simulink model "FCSMPC_double_vector_2025b"  (R2025b)
settings: Solver=FixedStepDiscrete  StartTime=0.0  StopTime=2  FixedStep=SimulinkTs  RelTol=1e-3
PreLoadFcn:
  | % Verzeichnis des Modells zum MATLAB-Pfad hinzufügen
  | modelDir = fileparts(get_param(bdroot, 'FileName'));
  | addpath(modelDir);
  | 
  | % Nur der Dateiname – kein Pfad!
  | set_param(bdroot, 'DataDictionary', 'FOC_params.sldd');
model workspace (MAT data in the model file):
  Np : Simulink.Parameter (value not decoded)
values from neighbouring files (symbols this model uses):
  Filter_Current_FilterTimeConst = 3.3333333333333335E-5    [FOC_params.sldd]
  Filter_Current_SensorTimeConst = 1.5915494309189535E-6    [FOC_params.sldd]
  FOC = evalin("base", "FOC")    [createFOC_SLDD.m]
  FOC_Control_Current_KIid = 10.0    [FOC_params.sldd]
  FOC_Control_Current_KIiq = 10.0    [FOC_params.sldd]
  FOC_Control_Current_KPid = 0.20418507462686566    [FOC_params.sldd]
  FOC_Control_Current_KPiq = 0.58674626865671642    [FOC_params.sldd]
  FOC_Control_Current_Krd = 0.8    [FOC_params.sldd]
  FOC_Control_Current_Krq = 0.8    [FOC_params.sldd]
  FOC_Control_Current_TclCur = 0.1    [FOC_params.sldd]
  FOC_Control_Current_Tnd = 0.1    [FOC_params.sldd]
  FOC_Control_Current_Tnq = 0.1    [FOC_params.sldd]
  FOC_Control_InverterVdc_V = 400.0    [FOC_params.sldd]
  FOC_Control_MotorImax_A = 650.0    [FOC_params.sldd]
  FOC_Control_MTPA_MTPV_nT_id_grid = -450.06704889786266 -439.56177000270145 -427.77784873303676 -416.66404703197372 -406.07553272717422 -395.15516533678584 -384.31176061747851 -374.03652088128132 -363.90551910193739 -353.79478643334204 -344.0221683092833 -334.51243453441936 -324.94614350292119 -315.21793409137081 -305.26543360965195 -295.21828280911944 -285.133916324101 -275.01232812136521 -264.86951532374729 -254.7797625148454 -244    [FOC_params.sldd]
  FOC_Control_MTPA_MTPV_nT_iq_grid = -449.09165648258488 -442.56958748923387 -437.25247759546528 -430.91792082419158 -423.83735797306491 -417.11730433547 -410.54064621830616 -403.71584331167304 -396.93611069310379 -390.15794305727007 -382.97216593027133 -375.44639668848538 -367.93447385667577 -360.57088856352266 -353.41289778449368 -346.34020584402072 -339.28416684923008 -332.22010880540631 -325.11927997033376 -317.92299905654966 -31    [FOC_params.sldd]
  FOC_Control_MTPA_MTPV_T_vec = -245.0 -240.0 -235.0 -230.0 -225.0 -220.0 -215.0 -210.0 -205.0 -200.0 -195.0 -190.0 -185.0 -180.0 -175.0 -170.0 -165.0 -160.0 -155.0 -150.0 -145.0 -140.0 -135.0 -130.0 -125.0 -120.0 -115.0 -110.0 -105.0 -100.0 -95.0 -90.0 -85.0 -80.0 -75.0 -70.0 -65.0 -60.0 -55.0 -50.0 -45.0 -40.0 -35.0 -30.0 -25.0 -20.0 -15.0 -10.0 -5.0 0.0 5.0 10.0 15.0 20.0 25.0 30.0 35.0 40.0 45.0 50.0 55.0 60.0 65.0 70.0 75.0    [FOC_params.sldd]
  FOC_Control_MTPA_MTPV_w_vec = 0.0 10.471975511965978 20.943951023931955 31.415926535897931 41.887902047863911 52.359877559829883 62.831853071795862 73.303828583761828 83.775804095727821 94.247779607693786 104.71975511965977 115.19173063162575 125.66370614359172 136.1356816555577 146.60765716752366 157.07963267948966 167.55160819145564 178.02358370342159 188.49555921538757 198.96753472735358 209.43951023931953 219.9114857512855    [FOC_params.sldd]
  FOC_Control_OpenLoop_Id_Ref_A = 0.0    [FOC_params.sldd]
  FOC_Control_OpenLoop_Iq_Ref_A = 0.0    [FOC_params.sldd]
  FOC_Control_OpenLoop_Ud_OpenLoop_V = 0.0    [FOC_params.sldd]
  FOC_Control_OpenLoop_Uq_OpenLoop_V = 0.0    [FOC_params.sldd]
  FOC_Control_RF_omegamech_rad_s = 3141.5926535897934    [FOC_params.sldd]
  FOC_Control_RF_RateCurrent_A = 500.0    [FOC_params.sldd]
  FOC_Control_RF_RateTrq_Nm = 500.0    [FOC_params.sldd]
  FOC_Control_theta_mechOffsetFix = 0.0    [FOC_params.sldd]
  FOC_Control_theta_mechOffsetTime = 0.0    [FOC_params.sldd]
  FOC_Control_TorqueRef_Nm = 10.0    [FOC_params.sldd]
  FOC_Control_Umax_V = 230.94010767585033    [FOC_params.sldd]
  FOC_Flag_ClosedLoopControl = 1.0    [FOC_params.sldd]
  FOC_Flag_ControlStrategy = 2.0    [FOC_params.sldd]
  FOC_Flag_PWMEnable = 1.0    [FOC_params.sldd]
  FOC_Flag_ResetControl = 0.0    [FOC_params.sldd]
  FOC_Flag_TorqueControl = 1.0    [FOC_params.sldd]
  FOC_LUT_DQLimiter_DQ_LUTScaling = 1.8749999999999995E-5    [FOC_params.sldd]
  FOC_PWM_AZSPWMMethod = 3.0    [FOC_params.sldd]
  FOC_PWM_HybridMode = 1.0    [FOC_params.sldd]
  FOC_PWM_LB1 = 0.5    [FOC_params.sldd]
  FOC_PWM_LB2 = 0.77    [FOC_params.sldd]
  FOC_PWM_PWMManuel = 1.0    [FOC_params.sldd]
  FOC_PWM_RSPWMMethod = 2.0    [FOC_params.sldd]
  FOC_PWM_UB1 = 0.66    [FOC_params.sldd]
  FOC_PWM_UB2 = 0.9    [FOC_params.sldd]
  FOC_SampleTime_TsCur = 0.0001    [FOC_params.sldd]
undefined symbols (not defined in the file or in its folder): dspblkCoreblockFVToolHelper, FCS, Filter, gcbh, Plant, SimulinkTs
libraries: hdlsllib x2, simulink x2, autolibfluxpmsm x1
(part 4 of 8)

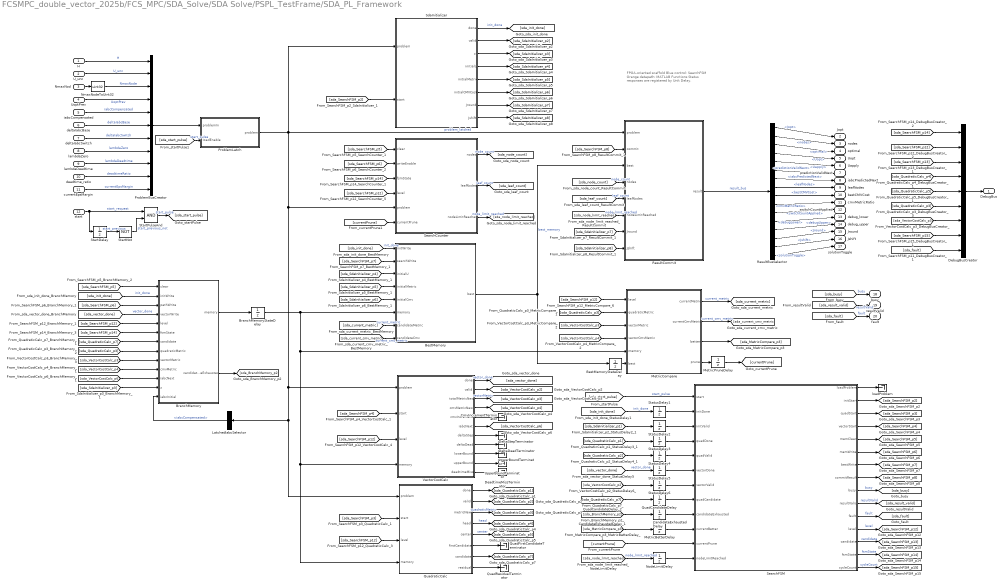
== system FCSMPC_double_vector_2025b/FCS_MPC/SDA_Solve/SDA Solve/PSPL_TestFrame/SDA_PL_Framework ==
  note: FPGA-oriented scaffold
      | Blue control: SearchFSM
      | Orange datapath: MATLAB Functions
      | Status responses are registered by Unit Delay.
  H : Inport
  U_unc : Inport  Port=2
  NmaxNod : Inport  Port=3
  UoptPrev : Inport  Port=4
  iabcCompensated : Inport  Port=5
  deltaIabcBase : Inport  Port=6
  deltaIabcSwitch : Inport  Port=7
  lambdaZero : Inport  Port=8
  lambdaDeadtime : Inport  Port=9
  deadtime_ratio : Inport  Port=10
  currentEpsMargin : Inport  Port=11
  start : Inport  Port=12  OutDataTypeStr=boolean
  BestMemory : MATLAB Function  TreatAsAtomicUnit=on
  BestMemoryStateDelay : UnitDelay  SampleTime=-1
  BranchMemory : MATLAB Function  TreatAsAtomicUnit=on
  BranchMemoryStateDelay : UnitDelay  SampleTime=-1
  CandidateExhaustedDelay : UnitDelay  InitialCondition=false  SampleTime=-1
  CmvIncrementTerminator : Terminator
  DeadtimeMissTerminator : Terminator
  DebugBusCreator : BusCreator  Inputs=9  OutDataTypeStr=Bus: SdaDebugBus
  DeltaDeadTerminator : Terminator
  DeltaStepTerminator : Terminator
  LatchedIabcSelector : BusSelector  OutputSignals=iabcCompensated
  LowerBoundTerminator : Terminator
  MetricBetterDelay : UnitDelay  InitialCondition=false  SampleTime=-1
  MetricCompare : MATLAB Function  TreatAsAtomicUnit=on
  MetricPruneDelay : UnitDelay  InitialCondition=false  SampleTime=-1
  NmaxNodeToUint32 : DataTypeConversion  OutDataTypeStr=uint32  SaturateOnIntegerOverflow=off  RndMeth=Floor
  NodeLimitDelay : UnitDelay  InitialCondition=false  SampleTime=-1
  ProblemBusCreator : BusCreator  Inputs=11  OutDataTypeStr=Bus: SdaProblemBus
  ProblemLatch : MATLAB Function  TreatAsAtomicUnit=on
  QuadCandidateDelay : UnitDelay  InitialCondition=false  SampleTime=-1
  QuadFirstCandidateTerminator : Terminator
  QuadResidualTerminator : Terminator
  QuadraticCalc : MATLAB Function  TreatAsAtomicUnit=on
  ResultBusSelector : BusSelector  OutputSignals=Jopt,nodes,optimal,Uopt,Uapply,predictionValidNext,iabcPredictedNext,leafNodes,bestCMVCost,cmvMetricRatio,switchCountApplied,debugLower,debugUpper,Jround,Jshift,solutionToggle
  ResultCommit : MATLAB Function  TreatAsAtomicUnit=on
  SdaInitializer : MATLAB Function  TreatAsAtomicUnit=on
  SearchCounter : MATLAB Function  TreatAsAtomicUnit=on
  SearchFSM : Stateflow chart  TreatAsAtomicUnit=on
  StartDelay : UnitDelay  InitialCondition=false  SampleTime=-1  HasFrameUpgradeWarning=on
  StartNot : Logic  Operator=NOT  AllPortsSameDT=off  OutDataTypeStr=boolean
  StartPulseAnd : Logic  AllPortsSameDT=off  OutDataTypeStr=boolean
  StatusDelay{1..6} (6 alike) : UnitDelay  InitialCondition=false  SampleTime=-1
  UpperBoundTerminator : Terminator
  VectorCostCalc : MATLAB Function  TreatAsAtomicUnit=on
  loadProblem : Terminator
  DebugBus : Outport  OutDataTypeStr=Bus: SdaDebugBus
  Jopt : Outport  Port=2
  nodes : Outport  Port=3
  optimal : Outport  Port=4
  Uopt : Outport  Port=5
  Uapply : Outport  Port=6
  predictionValidNext : Outport  Port=7
  iabcPredictedNext : Outport  Port=8
  leafNodes : Outport  Port=9
  bestCMVCost : Outport  Port=10
  cmvMetricRatio : Outport  Port=11
  switchCountApplied : Outport  Port=12
  debug_lower : Outport  Port=13
  debug_upper : Outport  Port=14
  Jround : Outport  Port=15
  Jshift : Outport  Port=16
  solutionToggle : Outport  Port=17
  busy : Outport  Port=18
  resultValid : Outport  Port=19
  fault : Outport  Port=20
  wires:
  NodeLimitDelay/1 -> SearchFSM/12(nodeLimitReached)
  MetricPruneDelay/1 -> [currentPrune]
  MetricBetterDelay/1 -> SearchFSM/10(currentBetter)
  BestMemoryStateDelay/1 -> MetricCompare/6(best)
  CandidateExhaustedDelay/1 -> SearchFSM/9(candidateExhausted)
  QuadCandidateDelay/1 -> SearchFSM/8(quadCandidate)
  BranchMemoryStateDelay/1 -> QuadraticCalc/4(memory), VectorCostCalc/4(memory), MetricCompare/5(memory), BestMemory/6(memory)
  NmaxNodeToUint32/1 -> ProblemBusCreator/3  "NmaxNode"
  NmaxNod/1 -> NmaxNodeToUint32/1
  DebugBusCreator/1 -> DebugBus/1
  SearchFSM/11(fault) -> [sda_fault]  "fault"
  StatusDelay6/1 -> SearchFSM/7(vectorValid)
  StatusDelay5/1 -> SearchFSM/6(vectorDone)
  StatusDelay4/1 -> SearchFSM/5(quadValid)
  StatusDelay3/1 -> SearchFSM/4(quadDone)
  StatusDelay2/1 -> SearchFSM/3(initValid)
  StatusDelay1/1 -> SearchFSM/2(initDone)
  ProblemBusCreator/1 -> ProblemLatch/1(problemIn)
  currentEpsMargin/1 -> ProblemBusCreator/11  "currentEpsMargin"
  deadtime_ratio/1 -> ProblemBusCreator/10  "deadtimeRatio"
  lambdaDeadtime/1 -> ProblemBusCreator/9  "lambdaDeadtime"
  lambdaZero/1 -> ProblemBusCreator/8  "lambdaZero"
  deltaIabcSwitch/1 -> ProblemBusCreator/7  "deltaIabcSwitch"
  deltaIabcBase/1 -> ProblemBusCreator/6  "deltaIabcBase"
  iabcCompensated/1 -> ProblemBusCreator/5  "iabcCompensated"
  UoptPrev/1 -> ProblemBusCreator/4  "UoptPrev"
  U_unc/1 -> ProblemBusCreator/2  "U_unc"
  H/1 -> ProblemBusCreator/1  "H"
  start/1 -> StartDelay/1, StartPulseAnd/1  "start_request"
  StartDelay/1 -> StartNot/1  "start_previous"
  StartNot/1 -> StartPulseAnd/2  "start_previous_not"
  StartPulseAnd/1 -> [sda_start_pulse]  "start_pulse"
  [sda_start_pulse] -> SearchFSM/1(start)  "start_pulse"
  ResultBusSelector/1 -> Jopt/1  "<Jopt>"
  ResultBusSelector/2 -> nodes/1  "<nodes>"
  ResultBusSelector/3 -> optimal/1  "<optimal>"
  ResultBusSelector/4 -> Uopt/1  "<Uopt>"
  ResultBusSelector/5 -> Uapply/1  "<Uapply>"
  ResultBusSelector/6 -> predictionValidNext/1  "<predictionValidNext>"
  ResultBusSelector/7 -> iabcPredictedNext/1  "<iabcPredictedNext>"
  ResultBusSelector/8 -> leafNodes/1  "<leafNodes>"
  ResultBusSelector/9 -> bestCMVCost/1  "<bestCMVCost>"
  ResultBusSelector/10 -> cmvMetricRatio/1  "<cmvMetricRatio>"
  ResultBusSelector/11 -> switchCountApplied/1  "<switchCountApplied>"
  ResultBusSelector/12 -> debug_lower/1  "<debugLower>"
  ResultBusSelector/13 -> debug_upper/1  "<debugUpper>"
  ResultBusSelector/14 -> Jround/1  "<Jround>"
  ResultBusSelector/15 -> Jshift/1  "<Jshift>"
  ResultBusSelector/16 -> solutionToggle/1  "<solutionToggle>"
  SearchFSM/9(busy) -> [sda_busy]  "busy"
  [sda_busy] -> busy/1  "busy"
  SearchFSM/10(resultValid) -> [sda_result_valid]  "resultValid"
  [sda_result_valid] -> resultValid/1  "resultValid"
  [sda_fault] -> fault/1  "fault"
  ProblemLatch/1(problem) -> QuadraticCalc/1(problem), LatchedIabcSelector/1, VectorCostCalc/1(problem), SearchCounter/5(problem), ResultCommit/1(problem), SdaInitializer/1(problem)  "problem_latched"
  BestMemory/1(best) -> ResultCommit/3(best), BestMemoryStateDelay/1  "best_memory"
  ResultCommit/1(result) -> ResultBusSelector/1  "result_bus"
  SdaInitializer/1(done) -> [sda_init_done]  "init_done"
  [sda_init_done] -> StatusDelay1/1  "init_done"
  [sda_init_done] -> BranchMemory/2(initWrite)  "init_done"
  [sda_init_done] -> BestMemory/1(initWrite)  "init_done"
  VectorCostCalc/1(done) -> [sda_vector_done]  "vector_done"
  [sda_vector_done] -> BranchMemory/4(vectorWrite)  "vector_done"
  [sda_vector_done] -> StatusDelay5/1  "vector_done"
  MetricCompare/1(currentMetric) -> [sda_current_metric]  "current_metric"
  [sda_current_metric] -> BestMemory/7(candidateMetric)  "current_metric"
  MetricCompare/2(currentCmvMetric) -> [sda_current_cmv_metric]  "current_cmv_metric"
  [sda_current_cmv_metric] -> BestMemory/8(candidateCmv)  "current_cmv_metric"
  SearchCounter/1(nodes) -> [sda_node_count]  "node_count"
  [sda_node_count] -> ResultCommit/4(nodes)  "node_count"
  SearchCounter/2(leafNodes) -> [sda_leaf_count]  "leaf_count"
  [sda_leaf_count] -> ResultCommit/5(leafNodes)  "leaf_count"
  SearchCounter/3(nodeLimitReached) -> [sda_node_limit_reached]  "node_limit_reached"
  [sda_node_limit_reached] -> ResultCommit/6(nodeLimitReached)  "node_limit_reached"
  [sda_node_limit_reached] -> NodeLimitDelay/1  "node_limit_reached"
  SearchFSM/1(loadProblem) -> loadProblem/1
  SearchFSM/2(initStart) -> [sda_SearchFSM_p2]
  [sda_SearchFSM_p2] -> SdaInitializer/2(start)
  SearchFSM/3(quadStart) -> [sda_SearchFSM_p3]
  [sda_SearchFSM_p3] -> QuadraticCalc/2(start)
  SearchFSM/4(vectorStart) -> [sda_SearchFSM_p4]
  [sda_SearchFSM_p4] -> VectorCostCalc/2(start)
  SearchFSM/5(memClear) -> [sda_SearchFSM_p5]
  [sda_SearchFSM_p5] -> SearchCounter/1(clear)
  [sda_SearchFSM_p5] -> BranchMemory/1(clear)
  SearchFSM/6(memWrite) -> [sda_SearchFSM_p6]
  [sda_SearchFSM_p6] -> BranchMemory/3(pathWrite)
  [sda_SearchFSM_p6] -> SearchCounter/2(writeEnable)
  SearchFSM/7(bestWrite) -> [sda_SearchFSM_p7]
  [sda_SearchFSM_p7] -> BestMemory/2(searchWrite)
  SearchFSM/8(commitResult) -> [sda_SearchFSM_p8]
  [sda_SearchFSM_p8] -> ResultCommit/2(commit)
  [sda_fault] -> DebugBusCreator/9
  SearchFSM/12(level) -> [sda_SearchFSM_p12]  "level"
  [sda_SearchFSM_p12] -> BranchMemory/5(level)
  [sda_SearchFSM_p12] -> DebugBusCreator/2
  [sda_SearchFSM_p12] -> QuadraticCalc/3(level)
  [sda_SearchFSM_p12] -> VectorCostCalc/3(level)
  [sda_SearchFSM_p12] -> SearchCounter/4(level)
  [sda_SearchFSM_p12] -> MetricCompare/1(level)
  SearchFSM/13(candidate) -> [sda_SearchFSM_p13]  "candidate"
  [sda_SearchFSM_p13] -> DebugBusCreator/3
  SearchFSM/14(fsmState) -> [sda_SearchFSM_p14]  "fsmState"
  [sda_SearchFSM_p14] -> SearchCounter/3(fsmState)
  [sda_SearchFSM_p14] -> DebugBusCreator/1
  [sda_SearchFSM_p14] -> BranchMemory/6(fsmState)
  SearchFSM/15(cycleCount) -> [sda_SearchFSM_p15]  "cycleCount"
  [sda_SearchFSM_p15] -> DebugBusCreator/8
  SdaInitializer/2(valid) -> [sda_SdaInitializer_p2]
  [sda_SdaInitializer_p2] -> StatusDelay2/1
  SdaInitializer/3(z) -> [sda_SdaInitializer_p3]
  [sda_SdaInitializer_p3] -> BranchMemory/12(z)
  SdaInitializer/4(initialU) -> [sda_SdaInitializer_p4]
  [sda_SdaInitializer_p4] -> BestMemory/3(initialU)
  SdaInitializer/5(initialMetric) -> [sda_SdaInitializer_p5]
  [sda_SdaInitializer_p5] -> BestMemory/4(initialMetric)
  SdaInitializer/6(initialCMVCost) -> [sda_SdaInitializer_p6]
  [sda_SdaInitializer_p6] -> BestMemory/5(initialCmv)
  SdaInitializer/7(Jround) -> [sda_SdaInitializer_p7]
  [sda_SdaInitializer_p7] -> ResultCommit/7(Jround)
  SdaInitializer/8(Jshift) -> [sda_SdaInitializer_p8]
  [sda_SdaInitializer_p8] -> ResultCommit/8(Jshift)
  QuadraticCalc/1(done) -> [sda_QuadraticCalc_p1]
  [sda_QuadraticCalc_p1] -> StatusDelay3/1
  QuadraticCalc/2(valid) -> [sda_QuadraticCalc_p2]
  [sda_QuadraticCalc_p2] -> StatusDelay4/1
  QuadraticCalc/3(metricNew) -> [sda_QuadraticCalc_p3]  "quadraticMetric"
  [sda_QuadraticCalc_p3] -> MetricCompare/2(quadraticMetric)
  [sda_QuadraticCalc_p3] -> BranchMemory/8(quadraticMetric)
  [sda_QuadraticCalc_p3] -> DebugBusCreator/6
  QuadraticCalc/4(head) -> [sda_QuadraticCalc_p4]  "head"
  [sda_QuadraticCalc_p4] -> DebugBusCreator/4
  QuadraticCalc/5(center) -> [sda_QuadraticCalc_p5]  "center"
  [sda_QuadraticCalc_p5] -> DebugBusCreator/5
  QuadraticCalc/6(firstCandidate) -> QuadFirstCandidateTerminator/1
  QuadraticCalc/7(candidate) -> [sda_QuadraticCalc_p7]
  [sda_QuadraticCalc_p7] -> BranchMemory/7(candidate)
  [sda_QuadraticCalc_p7] -> QuadCandidateDelay/1
  QuadraticCalc/8(residual) -> QuadResidualTerminator/1
  VectorCostCalc/2(valid) -> [sda_VectorCostCalc_p2]
  [sda_VectorCostCalc_p2] -> StatusDelay6/1
  VectorCostCalc/3(totalMetricNew) -> [sda_VectorCostCalc_p3]  "vectorMetric"
  [sda_VectorCostCalc_p3] -> DebugBusCreator/7
  [sda_VectorCostCalc_p3] -> MetricCompare/3(vectorMetric)
  [sda_VectorCostCalc_p3] -> BranchMemory/9(vectorMetric)
  VectorCostCalc/4(cmvMetricNew) -> [sda_VectorCostCalc_p4]
  [sda_VectorCostCalc_p4] -> BranchMemory/10(cmvMetric)
  [sda_VectorCostCalc_p4] -> MetricCompare/4(vectorCmvMetric)
  VectorCostCalc/5(cmvIncrement) -> CmvIncrementTerminator/1
  VectorCostCalc/6(iabcNext) -> [sda_VectorCostCalc_p6]
  [sda_VectorCostCalc_p6] -> BranchMemory/11(iabcNext)
  VectorCostCalc/7(deltaStep) -> DeltaStepTerminator/1
  VectorCostCalc/8(deltaDead) -> DeltaDeadTerminator/1
  VectorCostCalc/9(lowerBound) -> LowerBoundTerminator/1
  VectorCostCalc/10(upperBound) -> UpperBoundTerminator/1
  VectorCostCalc/11(deadtimeMiss) -> DeadtimeMissTerminator/1
  BranchMemory/1(memory) -> BranchMemoryStateDelay/1
  BranchMemory/2(candidateExhausted) -> [sda_BranchMemory_p2]
  [sda_BranchMemory_p2] -> CandidateExhaustedDelay/1
  MetricCompare/3(better) -> [sda_MetricCompare_p3]
  [sda_MetricCompare_p3] -> MetricBetterDelay/1
  MetricCompare/4(prune) -> MetricPruneDelay/1
  [currentPrune] -> SearchFSM/11(currentPrune)
  [currentPrune] -> SearchCounter/6(currentPrune)
  LatchedIabcSelector/1 -> BranchMemory/13(iabcInitial)  "<iabcCompensated>"
  [sda_start_pulse] -> ProblemLatch/2(loadEnable)  "start_pulse"

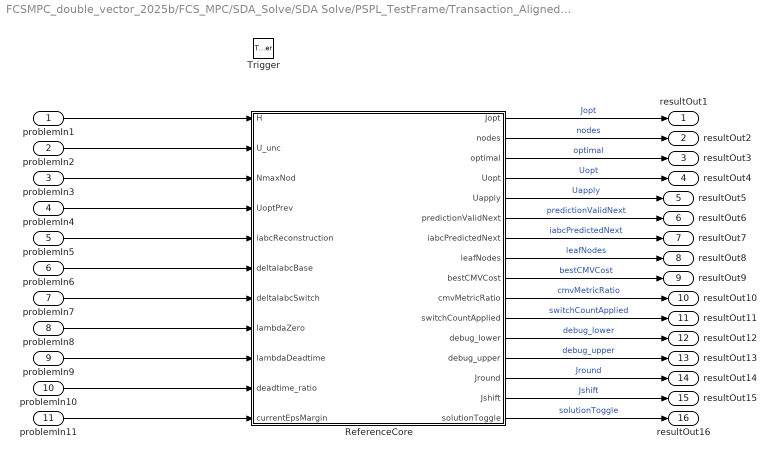
== system FCSMPC_double_vector_2025b/FCS_MPC/SDA_Solve/SDA Solve/PSPL_TestFrame/Transaction_Aligned_Reference ==
  problemIn1 : Inport
  problemIn2 : Inport  Port=2
  problemIn3 : Inport  Port=3
  problemIn4 : Inport  Port=4
  problemIn5 : Inport  Port=5
  problemIn6 : Inport  Port=6
  problemIn7 : Inport  Port=7
  problemIn8 : Inport  Port=8
  problemIn9 : Inport  Port=9
  problemIn10 : Inport  Port=10
  problemIn11 : Inport  Port=11
  Trigger : TriggerPort  VariantControl=(inherit)
  ReferenceCore : MATLAB Function  TreatAsAtomicUnit=on
  resultOut1 : Outport
  resultOut2 : Outport  Port=2
  resultOut3 : Outport  Port=3
  resultOut4 : Outport  Port=4
  resultOut5 : Outport  Port=5
  resultOut6 : Outport  Port=6
  resultOut7 : Outport  Port=7
  resultOut8 : Outport  Port=8
  resultOut9 : Outport  Port=9
  resultOut10 : Outport  Port=10
  resultOut11 : Outport  Port=11
  resultOut12 : Outport  Port=12
  resultOut13 : Outport  Port=13
  resultOut14 : Outport  Port=14
  resultOut15 : Outport  Port=15
  resultOut16 : Outport  Port=16
  wires:
  problemIn1/1 -> ReferenceCore/1(H)
  problemIn2/1 -> ReferenceCore/2(U_unc)
  problemIn3/1 -> ReferenceCore/3(NmaxNod)
  problemIn4/1 -> ReferenceCore/4(UoptPrev)
  problemIn5/1 -> ReferenceCore/5(iabcReconstruction)
  problemIn6/1 -> ReferenceCore/6(deltaIabcBase)
  problemIn7/1 -> ReferenceCore/7(deltaIabcSwitch)
  problemIn8/1 -> ReferenceCore/8(lambdaZero)
  problemIn9/1 -> ReferenceCore/9(lambdaDeadtime)
  problemIn10/1 -> ReferenceCore/10(deadtime_ratio)
  problemIn11/1 -> ReferenceCore/11(currentEpsMargin)
  ReferenceCore/1(Jopt) -> resultOut1/1  "Jopt"
  ReferenceCore/2(nodes) -> resultOut2/1  "nodes"
  ReferenceCore/3(optimal) -> resultOut3/1  "optimal"
  ReferenceCore/4(Uopt) -> resultOut4/1  "Uopt"
  ReferenceCore/5(Uapply) -> resultOut5/1  "Uapply"
  ReferenceCore/6(predictionValidNext) -> resultOut6/1  "predictionValidNext"
  ReferenceCore/7(iabcPredictedNext) -> resultOut7/1  "iabcPredictedNext"
  ReferenceCore/8(leafNodes) -> resultOut8/1  "leafNodes"
  ReferenceCore/9(bestCMVCost) -> resultOut9/1  "bestCMVCost"
  ReferenceCore/10(cmvMetricRatio) -> resultOut10/1  "cmvMetricRatio"
  ReferenceCore/11(switchCountApplied) -> resultOut11/1  "switchCountApplied"
  ReferenceCore/12(debug_lower) -> resultOut12/1  "debug_lower"
  ReferenceCore/13(debug_upper) -> resultOut13/1  "debug_upper"
  ReferenceCore/14(Jround) -> resultOut14/1  "Jround"
  ReferenceCore/15(Jshift) -> resultOut15/1  "Jshift"
  ReferenceCore/16(solutionToggle) -> resultOut16/1  "solutionToggle"

== stateflow chart FCSMPC_double_vector_2025b/FCS_MPC/CurrentRefCalc/Current_RateLimiter/RateLimiter1 ==
  settings: updateMethod=DISCRETE  sampleTime=FOC.SampleTime.TsSpeed
  state IDLE
  state Rising
    entry:  y =  fi(y_prev +dT * R, 1, 32, 18);
    exit: y_prev = y;
  state Falling
    entry:  y = fi(y_prev+dT * F, 1, 32, 18);
    exit: y_prev = y;
  state Directpassage
    entry:  y = u;
    exit: y_prev = y;
  (default) -> IDLE
  IDLE -> (junction 22)
  (junction 22) -> Rising [order 1] : [(u-y_prev)/dT>=R]
  (junction 22) -> Falling [order 2] : [(u-y_prev)/dT<=F]
  Rising -> (junction 22)
  Falling -> (junction 22)
  Directpassage -> (junction 22)
  (junction 22) -> Directpassage [order 3] : [(u-y_prev)/dT<R && (u-y_prev)/dT>F]
  data: u input fixdt(1,32,18); R input fixdt(1,32,18); F input fixdt(1,32,18); dT constant fixdt(1,32,18) size=1 =FOC.SampleTime.TsSpeed; y output fixdt(1,32,18); y_prev local fixdt(1,32,18) =0

== stateflow chart FCSMPC_double_vector_2025b/FCS_MPC/CurrentRefCalc/RateLimiter ==
  settings: updateMethod=DISCRETE  sampleTime=FOC.SampleTime.TsSpeed
  state IDLE
  state Rising
    entry:  y =  fi(y_prev +dT * R, 1, 32, 18);
    exit: y_prev = y;
  state Falling
    entry:  y = fi(y_prev+dT * F, 1, 32, 18);
    exit: y_prev = y;
  state Directpassage
    entry:  y = u;
    exit: y_prev = y;
  (default) -> IDLE
  IDLE -> (junction 22)
  (junction 22) -> Rising [order 1] : [(u-y_prev)/dT>=R]
  (junction 22) -> Falling [order 2] : [(u-y_prev)/dT<=F]
  Rising -> (junction 22)
  Falling -> (junction 22)
  Directpassage -> (junction 22)
  (junction 22) -> Directpassage [order 3] : [(u-y_prev)/dT<R && (u-y_prev)/dT>F]
  data: u input fixdt(1,32,18); R input fixdt(1,32,18); F input fixdt(1,32,18); dT constant fixdt(1,32,18) size=1 =FOC.SampleTime.TsSpeed; y output fixdt(1,32,18); y_prev local fixdt(1,32,18) =0

== matlab function FCSMPC_double_vector_2025b/FCS_MPC/SDA_Solve/SDA Solve/PSPL_TestFrame/SDA_PL_Framework/BestMemory ==
  data: initWrite input boolean size=[1 1]; searchWrite input boolean size=[1 1]; best output Bus: SdaBestBus size=[1 1]; initialU input double size=[15 1]; initialMetric input double size=[1 1]; initialCmv input double size=[1 1]; memory input Bus: SdaMemoryBus size=[1 1]; candidateMetric input double size=[1 1]; candidateCmv input double size=[1 1]
function best = BestMemory(initWrite,searchWrite,initialU,initialMetric,initialCmv,memory,candidateMetric,candidateCmv)
%#codegen
persistent state
if isempty(state)
 state.bestU=false(15,1); state.bestMetric=realmax;
 state.bestCMVCost=0.0; state.bestValid=false;
end
if initWrite
 state.bestU=initialU>0.5; state.bestMetric=initialMetric;
 state.bestCMVCost=initialCmv; state.bestValid=isfinite(initialMetric);
elseif searchWrite&&candidateMetric<state.bestMetric
 state.bestU=memory.Uwork; state.bestMetric=candidateMetric;
 state.bestCMVCost=candidateCmv; state.bestValid=isfinite(candidateMetric);
end
best=state;
end

== stateflow chart FCSMPC_double_vector_2025b/Plant_PMSM_INV/RateLimiter ==
  settings: updateMethod=DISCRETE  sampleTime=FOC.SampleTime.TsSpeed
  state IDLE
  state Rising
    entry:  y = dT*R+y_prev;
    exit: y_prev = y;
  state Falling
    entry:  y = dT*F+y_prev;
    exit: y_prev = y;
  state Directpassage
    entry:  y = u;
    exit: y_prev = y;
  (default) -> IDLE
  IDLE -> (junction 22)
  (junction 22) -> Rising [order 1] : [(u-y_prev)/dT>=R]
  (junction 22) -> Falling [order 2] : [(u-y_prev)/dT<=F]
  Rising -> (junction 22)
  Falling -> (junction 22)
  Directpassage -> (junction 22)
  (junction 22) -> Directpassage [order 3] : [(u-y_prev)/dT<R && (u-y_prev)/dT>F]
  data: u input; R input; F input; dT constant double size=1 =FOC.SampleTime.TsSpeed; y output; y_prev local double =0

== matlab function FCSMPC_double_vector_2025b/FCS_MPC/SDA_Solve/SDA Solve/PSPL_TestFrame/Transaction_Aligned_Reference/ReferenceCore ==
  data: H input double size=[15 15]; Jopt output double size=[1 1]; U_unc input double size=[15 1]; NmaxNod input double size=[1 1]; UoptPrev input double size=[15 1]; iabcReconstruction input double size=[3 1]; deltaIabcBase input double size=[3 1]; deltaIabcSwitch input double size=[3 3]; lambdaZero input double size=[1 1]; lambdaDeadtime input double size=[1 1]; deadtime_ratio input double size=[1 1]; currentEpsMargin input double size=[1 1]; nodes output double size=[1 1]; optimal output boolean size=[1 1]; Uopt output double size=[15 1]; Uapply output double size=[6 1]; predictionValidNext output boolean size=[1 1]; iabcPredictedNext output double size=[3 1]; leafNodes output double size=[1 1]; bestCMVCost output double size=[1 1]; cmvMetricRatio output double size=[1 1]; switchCountApplied output double size=[1 1]; debug_lower output double size=[3 1]; debug_upper output double size=[3 1]; Jround output double size=[1 1]; Jshift output double size=[1 1]; solutionToggle output boolean size=[1 1]
function [Jopt, nodes, optimal, Uopt, Uapply, ...
    predictionValidNext,iabcPredictedNext, ...
    leafNodes, bestCMVCost, cmvMetricRatio, switchCountApplied, ...
    debug_lower, debug_upper, Jround, Jshift, solutionToggle] = ...
    SDA_Solve_Synchronized(H, U_unc, NmaxNod, UoptPrev, ...
    iabcReconstruction, deltaIabcBase, deltaIabcSwitch, ...
    lambdaZero, lambdaDeadtime, deadtime_ratio, currentEpsMargin)
%SDA_SOLVE Independent double-vector SDA MATLAB Function module.
% The first five ports follow FCSMPC_IdealSDA. Feed Uopt back to UoptPrev
% through a Unit Delay initialized with zeros(15,1). UapplyFirst and
% UapplySecond are applied successively for half an external period each.

Np = 5;
nu = 3;
n = numel(U_unc);

Ubar = H*U_unc;
uprev = UoptPrev(4:6);
deadtimeRatio = deadtime_ratio;

Uround = min(max(round(U_unc),0.0),1.0);
Ushift = zeros(n,1);
Ushift(1:n-nu) = UoptPrev(nu+1:n);
Ushift(n-nu+1:n) = UoptPrev(n-nu+1:n);
Jround = norm(H*(Uround-U_unc),2)^2;
Jshift = norm(H*(Ushift-U_unc),2)^2;
if Jshift < Jround
    Uini = Ushift;
else
    Uini = Uround;
end

bestCMVCost = sequence_cmv_cost_predicted( ...
    Uini,uprev,iabcReconstruction,Np,nu, ...
    deltaIabcBase,deltaIabcSwitch,lambdaZero,lambdaDeadtime, ...
    deadtimeRatio,currentEpsMargin);
bestMetric = norm(H*(Uini-U_unc),2)^2+bestCMVCost;
Uopt = Uini;

U = zeros(n,1);
kidx = ones(n,1);
d2s = zeros(n+1,1);
cmvD2s = zeros(n+1,1);
iabcPrediction = zeros(3,Np+1);
iabcPrediction(:,1) = iabcReconstruction;
nodes = 0;
leafNodes = 0;
optimal = true;
i = 1;

while i >= 1
    if kidx(i) > 2
        kidx(i) = 1;
        i = i-1;
        continue;
    end
    head = 0.0;
    if i > 1
        head = H(i,1:i-1)*U(1:i-1);
    end
    center = (Ubar(i)-head)/H(i,i);
    if center <= 0.5
        firstCandidate = 0.0;
    else
        firstCandidate = 1.0;
    end
    if kidx(i) == 1
        candidate = firstCandidate;
    else
        candidate = 1.0-firstCandidate;
    end
    kidx(i) = kidx(i)+1;
    U(i) = candidate;
    nodes = nodes+1;
    if NmaxNod > 0 && nodes > NmaxNod
        optimal = false;
        break;
    end

    residual = Ubar(i)-head-H(i,i)*candidate;
    metricNew = d2s(i)+residual*residual;
    cmvMetricNew = cmvD2s(i);
    if mod(i,nu) == 0
        predictionStep = i/nu;
        blockStart = i-nu+1;
        uCurrent = U(blockStart:i);
        if predictionStep == 1
            uPrevious = uprev;
        else
            uPrevious = U(blockStart-nu:blockStart-1);
        end
        iabcBeforeSwitch = iabcPrediction(:,predictionStep);
        [deltaStep,deltaDead] = deadtime_corrected_current_step( ...
            uPrevious,uCurrent,iabcBeforeSwitch, ...
            deltaIabcBase,deltaIabcSwitch,deadtimeRatio,currentEpsMargin);
        cmvIncrement = cmv_cost( ...
            uPrevious,uCurrent,iabcBeforeSwitch,deltaDead, ...
            lambdaZero,lambdaDeadtime,currentEpsMargin);
        metricNew = metricNew+cmvIncrement;
        cmvMetricNew = cmvMetricNew+cmvIncrement;
        iabcPrediction(:,predictionStep+1) = iabcBeforeSwitch+deltaStep;
    end
    if metricNew > bestMetric
        continue;
    end
    if i == n
        leafNodes = leafNodes+1;
        if metricNew < bestMetric
            bestMetric = metricNew;
            Uopt = U;
            bestCMVCost = cmvMetricNew;
        end
    else
        d2s(i+1) = metricNew;
        cmvD2s(i+1) = cmvMetricNew;
        i = i+1;
        kidx(i) = 1;
    end
end

if ~isfinite(bestMetric)
    Uopt = repmat(uprev,Np,1);
end

Uapply = Uopt(1:6);
UapplyFirst = Uopt(1:3);
UapplySecond = Uopt(4:6);

[deltaFirst,~] = deadtime_corrected_current_step( ...
    uprev,UapplyFirst,iabcReconstruction, ...
    deltaIabcBase,deltaIabcSwitch, ...
    deadtimeRatio,currentEpsMargin);
iabcAfterFirst = iabcReconstruction + deltaFirst;

[deltaSecond,~] = deadtime_corrected_current_step( ...
    UapplyFirst,UapplySecond,iabcAfterFirst, ...
    deltaIabcBase,deltaIabcSwitch,deadtimeRatio,currentEpsMargin);
iabcPredictedNext = iabcAfterFirst+deltaSecond;

switchCountApplied = sum(abs(UapplyFirst-uprev))+ ...
    sum(abs(UapplySecond-UapplyFirst));
Jopt = bestMetric;
if Jopt > eps
    cmvMetricRatio = bestCMVCost/Jopt;
else
    cmvMetricRatio = 0.0;
end
[~,debugDeltaDead] = deadtime_corrected_current_step( ...
    uprev,UapplyFirst,iabcReconstruction,deltaIabcBase,deltaIabcSwitch, ...
    deadtimeRatio,currentEpsMargin);
[~,debug_lower,debug_upper] = cmv_cost( ...
    uprev,UapplyFirst,iabcReconstruction,debugDeltaDead, ...
    lambdaZero,lambdaDeadtime,currentEpsMargin);
predictionValidNext = true;

% Toggle once after every completed SDA solution. The downstream switch
% detects this edge and explicitly restarts from the first vector.
persistent solutionToggleState
if isempty(solutionToggleState)
    solutionToggleState = false;
end
solutionToggleState = ~solutionToggleState;
solutionToggle = solutionToggleState;
end

function [deltaStep,deltaDead] = deadtime_corrected_current_step( ...
    uPrevious,uCurrent,iabcBeforeSwitch, ...
    deltaBase,deltaSwitch,deadtimeRatio,currentEps)
uDead = uCurrent;
changed = (uPrevious ~= uCurrent);
signEps = 0.1*currentEps;
for phase = 1:3
    if ~changed(phase)
        continue;
    end
    iPhase = iabcBeforeSwitch(phase);
    if iPhase >= signEps
        uDead(phase) = 0.0;
    elseif iPhase <= -signEps
        uDead(phase) = 1.0;
    else
        uDead(phase) = 0.5*(1.0-iPhase/signEps);
    end
end
uEffective = deadtimeRatio*uDead+(1.0-deadtimeRatio)*uCurrent;
deltaDead = deadtimeRatio*(deltaBase+deltaSwitch*uDead);
deltaStep = deltaBase+deltaSwitch*uEffective;
end

function [penalty,lowerBound,upperBound] = cmv_cost( ...
    uPrevious,uCurrent,iabcBeforeSwitch,deltaDead, ...
    lambdaZero,lambdaDeadtime,currentEpsMargin)
penalty = 0.0;
iabcDeadEnd = iabcBeforeSwitch+deltaDead;
lowerBound = min(iabcBeforeSwitch,iabcDeadEnd)-currentEpsMargin;
upperBound = max(iabcBeforeSwitch,iabcDeadEnd)+currentEpsMargin;
uncertain = (lowerBound <= 0.0) & (upperBound >= 0.0);
if all(uCurrent == 0.0) || all(uCurrent == 1.0)
    penalty = penalty+lambdaZero;
end
changed = (uPrevious ~= uCurrent);
if sum(changed) ~= 2
    return;
end
canBeZero = false(3,1);
canBeOne = false(3,1);
for phase = 1:3
    if ~changed(phase)
        canBeZero(phase) = (uPrevious(phase) == 0.0);
        canBeOne(phase) = (uPrevious(phase) == 1.0);
    elseif uncertain(phase)
        canBeZero(phase) = true;
        canBeOne(phase) = true;
    elseif iabcDeadEnd(phase) > 0.0
        canBeZero(phase) = true;
    else
        canBeOne(phase) = true;
    end
end
if all(canBeZero) || all(canBeOne)
    penalty = penalty+lambdaDeadtime;
end
end

function totalPenalty = sequence_cmv_cost_predicted( ...
    U,uprev,iabcInitial,Np,nu,deltaBase,deltaSwitch, ...
    lambdaZero,lambdaDeadtime,deadtimeRatio,currentEpsMargin)
totalPenalty = 0.0;
uPrevious = uprev;
iabcBeforeSwitch = iabcInitial;
for step = 1:Np
    rows = (step-1)*nu+(1:nu);
    uCurrent = U(rows);
    [deltaStep,deltaDead] = deadtime_corrected_current_step( ...
        uPrevious,uCurrent,iabcBeforeSwitch,deltaBase,deltaSwitch, ...
        deadtimeRatio,currentEpsMargin);
    totalPenalty = totalPenalty+cmv_cost( ...
        uPrevious,uCurrent,iabcBeforeSwitch,deltaDead, ...
        lambdaZero,lambdaDeadtime,currentEpsMargin);
    iabcBeforeSwitch = iabcBeforeSwitch+deltaStep;
    uPrevious = uCurrent;
end
end

== matlab function FCSMPC_double_vector_2025b/Plant_PMSM_INV/MATLAB Function ==
  data: g_H input; g_L input; v_ph output; i_ph input; U_dc input; v_cmv output; v_legN output; v_err output
function [v_ph, v_cmv, v_legN, v_err] = inverter_model_gates(g_H, g_L, i_ph, U_dc)
%#codegen
% INVERTER_MODEL_GATES  Zweistufiger B6-Wechselrichter, zustandslos.
%
%   Erwartet die sechs Gate-Signale, in denen die Totzeit bereits
%   enthalten ist (waehrend der Totzeit sind g_H(k) und g_L(k) beide 0).
%   Dadurch benoetigt der Block keinen internen Zaehler und keine
%   Rueckfuehrung -- er ist rein kombinatorisch.
%
%   Eingaenge:
%     g_H   3x1 logical  Gate oberer Schalter je Bein
%     g_L   3x1 logical  Gate unterer Schalter je Bein
%     i_ph  3x1 double   Phasenstroeme [A], Zaehlpfeil aus dem Bein heraus
%     U_dc  1x1 double   Zwischenkreisspannung [V]
%
%   Ausgaenge:
%     v_ph   3x1 double  Strangspannungen gegen Sternpunkt [V]
%     v_cmv  1x1 double  Gleichtaktspannung gegen DC-Mittelpunkt [V]
%     v_legN 3x1 double  Beinpotenziale gegen DC-Minus [V]
%     v_err  3x1 double  Abweichung vom idealen Kommandowert [V] (Diagnose)

% ------------------------------------------------------------------
% Parameter
% ------------------------------------------------------------------
U_CE = 1.5;    % IGBT-Durchlassspannung [V]  (0 -> idealer Schalter)
U_F  = 1.2;    % Diodenflussspannung [V]     (0 -> ideale Diode)

v_legN    = zeros(3,1);
v_leg_cmd = zeros(3,1);

for k = 1:3

    ik = i_ph(k);
    hi = g_H(k);
    lo = g_L(k);

    if hi && ~lo
        % ===== Oberer Schalter eingeschaltet =====
        if ik >= 0
            v_legN(k) = U_dc - U_CE;    % oberer IGBT leitet
        else
            v_legN(k) = U_dc + U_F;     % obere Diode leitet
        end
        v_leg_cmd(k) = U_dc;

    elseif ~hi && lo
        % ===== Unterer Schalter eingeschaltet =====
        if ik > 0
            v_legN(k) = -U_F;           % untere Diode leitet
        else
            v_legN(k) = U_CE;           % unterer IGBT leitet
        end
        v_leg_cmd(k) = 0;

    elseif ~hi && ~lo
        % ===== TOTZEIT: beide Gates aus, Diode entscheidet =====
        if ik > 0
            v_legN(k) = -U_F;           % untere Freilaufdiode
            v_leg_cmd(k) = 0;
        else
            v_legN(k) = U_dc + U_F;     % obere Freilaufdiode
            v_leg_cmd(k) = U_dc;
        end

    else
        % ===== Beide Gates an: Bruecken-Kurzschluss =====
        % Physikalisch ein Fehlerfall. Hier als halbe Zwischenkreis-
        % spannung modelliert, damit die Simulation nicht divergiert.
        v_legN(k)    = 0.5 * U_dc;
        v_leg_cmd(k) = 0.5 * U_dc;
    end
end

% ------------------------------------------------------------------
% Sternpunktpotenzial, Strangspannungen, Gleichtaktspannung
% ------------------------------------------------------------------
% Symmetrische Last mit isoliertem Sternpunkt: Summe der Strangspannungen
% ist null, daraus folgt v_nN als Mittelwert der Beinpotenziale.
v_nN  = (v_legN(1) + v_legN(2) + v_legN(3)) / 3;

v_ph  = v_legN - v_nN;              % treiben die Maschine
v_cmv = v_nN - 0.5 * U_dc;          % gegen DC-Mittelpunkt

v_err = v_legN - v_leg_cmd;         % Diagnose: Abweichung vom Ideal

end

== matlab function FCSMPC_double_vector_2025b/FCS_MPC/Double_Vector_Switch/MATLAB Function ==
  data: UapplyFirst input; U_apply output; UapplySecond input; solutionToggle input; selectedHalf output; newSolutionDetected output
function [U_apply, selectedHalf, newSolutionDetected] = ...
    double_vector_switch_synchronized( ...
    UapplyFirst, UapplySecond, solutionToggle)
%DOUBLE_VECTOR_SWITCH_SYNCHRONIZED Apply a new vector pair in fixed order.
% solutionToggle changes once whenever SDA_Solve_Synchronized finishes.
% Its edge resets the sequence to UapplyFirst. The next invocation applies
% UapplySecond. Further invocations hold UapplySecond until a new solution.
%
% Diagnostic outputs:
%   selectedHalf        uint8(1): first vector; uint8(2): second vector
%   newSolutionDetected true on the call accepting a new SDA result

persistent lastSolutionToggle
persistent secondVectorPending

currentSolutionToggle = logical(solutionToggle);
if isempty(lastSolutionToggle)
    % Treat the first invocation as the arrival of a new SDA solution.
    lastSolutionToggle = ~currentSolutionToggle;
    secondVectorPending = false;
end

newSolutionDetected = (currentSolutionToggle ~= lastSolutionToggle);

if newSolutionDetected
    U_apply = UapplyFirst;
    selectedHalf = uint8(1);
    secondVectorPending = true;
    lastSolutionToggle = currentSolutionToggle;
elseif secondVectorPending
    U_apply = UapplySecond;
    selectedHalf = uint8(2);
    secondVectorPending = false;
else
    % Do not restart an old vector pair if this task runs unexpectedly.
    U_apply = UapplySecond;
    selectedHalf = uint8(2);
end

end
